simulink model "sixdof"  (Simulink 4.00)
settings: Solver=ode45  StartTime=0.0  StopTime=100  RelTol=1e-3
libraries: aerospace x3, simulink_extras x3, simulink3 x1
settings Model: Creator=mcar  LastModifiedBy=mcar  BlockReductionOpt=off

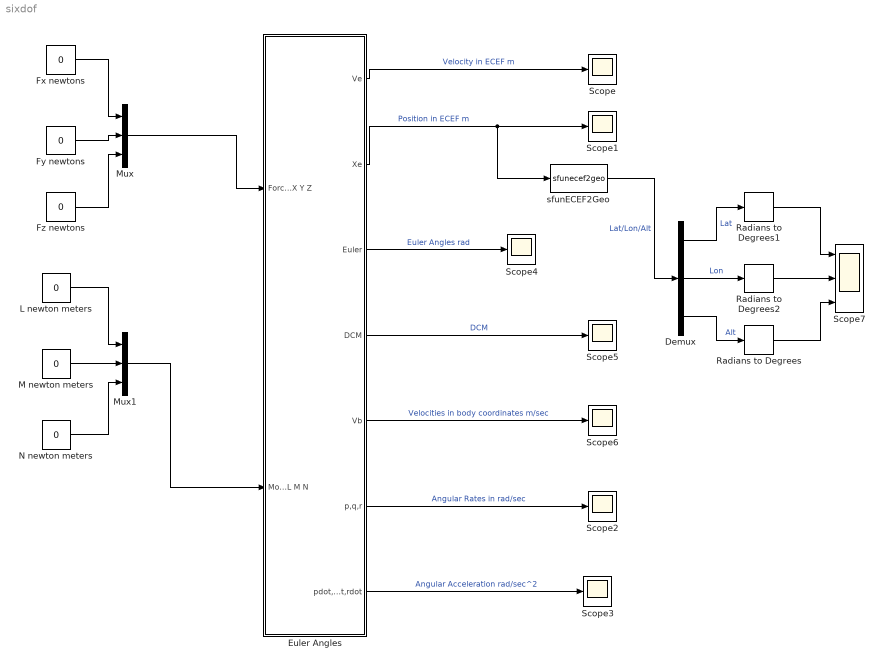
== system sixdof ==
  Demux : Demux  Outputs=3  BusSelectionMode=off
  Euler Angles : Subsystem  AncestorBlock=aerospace/6DoF/Euler Angles  mask{xme_0=[6.378137e6 0 0], Vm_0=[1 1 0], eul_0=[0 0 0], pm_0=[0 0 0], Mass=1.0, Inertia=[1.0 0 0;0 1.0 0;0 0 1.0]}
      mask prompts: xme_0 "Initial Inertial Position [Xe,Ye,Ze]"; Vm_0 "Initial Body Velocity [U,v,w]"; eul_0 "Initial Euler Orientation [roll, pitch, yaw]"; pm_0 "Initial Body Rates [p,q,r]"; Mass "Mass of body"; Inertia "Inertia Matrix"
      mask help: Euler Angles
      settings: RTWFcnNameOpts=Auto  RTWFileNameOpts=Auto
      mask Display: disp('Euler\nAngles')
  Fx newtons : Constant  Value=0
  Fy newtons : Constant  Value=0
  Fz newtons : Constant  Value=0
  L newton meters : Constant  Value=0
  M newton meters : Constant  Value=0
  Mux : Mux  Inputs=3
  Mux1 : Mux  Inputs=3
  N newton meters : Constant  Value=0
  Radians to Degrees : simulink_extras/Transformations/Radians to Degrees
  Radians to Degrees1 : simulink_extras/Transformations/Radians to Degrees
  Radians to Degrees2 : simulink_extras/Transformations/Radians to Degrees
  Scope{,1..6} (7 alike) : Scope
      Scope settings: TimeRange=auto  YMin=-5  YMax=5  SaveToWorkspace=off  SaveName=ScopeData  LimitDataPoints=on  MaxDataPoints=5000
      Scope1 settings: TickLabels=on  TimeRange=auto  YMin=-5  YMax=5  SaveToWorkspace=off  LimitDataPoints=on  MaxDataPoints=5000
      Scope2 settings: TimeRange=auto  YMin=-5  YMax=5  SaveToWorkspace=off  SaveName=ScopeData2  LimitDataPoints=on  MaxDataPoints=5000
      Scope3 settings: TimeRange=auto  YMin=-5  YMax=5  SaveToWorkspace=off  SaveName=ScopeData3  LimitDataPoints=on  MaxDataPoints=5000
      Scope4 settings: TickLabels=on  TimeRange=auto  YMin=-5  YMax=5  SaveToWorkspace=off  SaveName=ScopeData4  LimitDataPoints=on  MaxDataPoints=5000
      Scope5 settings: TickLabels=on  TimeRange=auto  YMin=-5  YMax=5  SaveToWorkspace=off  SaveName=ScopeData5  LimitDataPoints=on  MaxDataPoints=5000
      Scope6 settings: TickLabels=on  TimeRange=auto  YMin=-5  YMax=5  SaveToWorkspace=off  SaveName=ScopeData6  LimitDataPoints=on  MaxDataPoints=5000
  Scope7 : Scope  NumInputPorts=3
      settings: TickLabels=on  TimeRange=auto  YMin=-5~-5~-5  YMax=5~5~5  SaveToWorkspace=off  SaveName=ScopeData7  LimitDataPoints=on  MaxDataPoints=5000
  sfunECEF2Geo : S-Function  FunctionName=sfunecef2geo  PortCounts=[]  SFunctionModules=''
  wires:
  Mux/1 -> Euler Angles/1(Forces X Y Z)
  Fz newtons/1 -> Mux/3
  Fy newtons/1 -> Mux/2
  Fx newtons/1 -> Mux/1
  Mux1/1 -> Euler Angles/2(Moments L M N)
  N newton meters/1 -> Mux1/3
  M newton meters/1 -> Mux1/2
  L newton meters/1 -> Mux1/1
  Euler Angles/7(pdot,qdot,rdot) -> Scope3/1  "Angular Acceleration rad/sec^2"
  Euler Angles/6(p,q,r) -> Scope2/1  "Angular Rates in rad/sec"
  Euler Angles/2(Xe) -> Scope1/1, sfunECEF2Geo/1  "Position in ECEF m"
  Euler Angles/1(Ve) -> Scope/1  "Velocity in ECEF m"
  Euler Angles/3(Euler) -> Scope4/1  "Euler Angles rad"
  Euler Angles/5(Vb) -> Scope6/1  "Velocities in body coordinates m/sec"
  Euler Angles/4(DCM) -> Scope5/1  "DCM"
  sfunECEF2Geo/1 -> Demux/1  "Lat/Lon/Alt"
  Demux/1 -> Radians to Degrees1/1  "Lat"
  Demux/2 -> Radians to Degrees2/1  "Lon"
  Demux/3 -> Radians to Degrees/1  "Alt"
  Radians to Degrees1/1 -> Scope7/1
  Radians to Degrees2/1 -> Scope7/2
  Radians to Degrees/1 -> Scope7/3

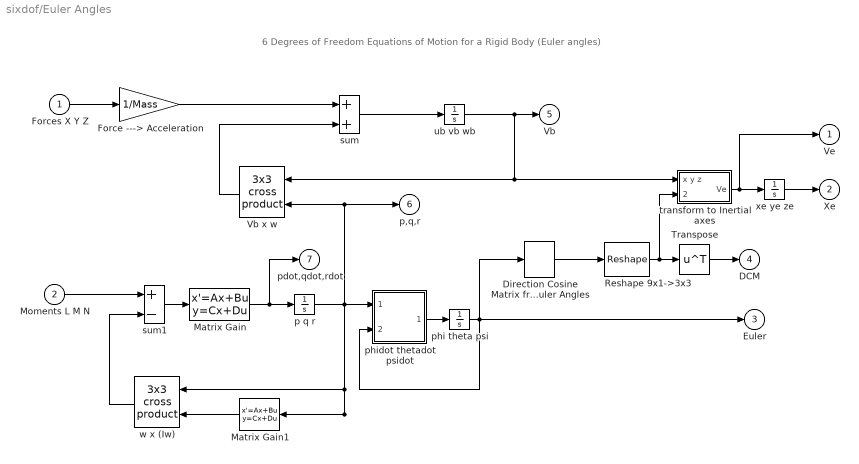
== system sixdof/Euler Angles ==
  note: 6 Degrees of Freedom Equations of Motion for a Rigid Body
      | (Euler angles)
  Forces X Y Z : Inport  Port=1
  Moments L M N : Inport  Port=2
  Direction Cosine Matrix from Euler Angles : aerospace/Axes Transformations/Direction Cosine Matrix from Euler Angles
  Force ---> Acceleration : Gain  Gain=1/Mass  Multiplication=Element-wise(K.*u)  SaturateOnIntegerOverflow=on
  Matrix Gain : StateSpace  A=[]  B=[]  C=[]  D=K  X0=0  Realization=auto  AbsoluteTolerance=auto  mask(Matrix Gain){@1=inv(Inertia)}
      mask prompts: @1 "Gain matrix:"
      mask help: Matrix Gain.
      mask init:
      | K = @1;
      mask Help: Multiplies input vector by entered matrix to produce output vector (y=Au).
      mask Display: disp('Inertia^(-1)')
  Matrix Gain1 : StateSpace  Orientation=left  A=[]  B=[]  C=[]  D=K  X0=0  Realization=auto  AbsoluteTolerance=auto  mask(Matrix Gain){@1=Inertia}
      mask prompts: @1 "Gain matrix:"
      mask help: Matrix Gain.
      mask init:
      | K = @1;
      mask Help: Multiplies input vector by entered matrix to produce output vector (y=Au).
      mask Display: disp('Inertia')
  Reshape 9x1->3x3 : simulink3/Signals & Systems/Reshape  OutputDimensionality=Customize  OutputDimensions=[3,3]
  Transpose : Math  Operator=transpose  OutputSignalType=auto
  Vb x w : aerospace/Axes Transformations/3x3 cross product  Orientation=left
  p q r : Integrator  ExternalReset=none  InitialConditionSource=internal  InitialCondition=pm_0  LimitOutput=off  UpperSaturationLimit=inf  LowerSaturationLimit=-inf  ShowSaturationPort=off  ShowStatePort=off  AbsoluteTolerance=auto
  phi theta psi : Integrator  ExternalReset=none  InitialConditionSource=internal  InitialCondition=eul_0  LimitOutput=off  UpperSaturationLimit=inf  LowerSaturationLimit=-inf  ShowSaturationPort=off  ShowStatePort=off  AbsoluteTolerance=auto
  phidot thetadot psidot : Subsystem
      settings: RTWFcnNameOpts=Auto  RTWFileNameOpts=Auto
  sum : Sum  Inputs=++  SaturateOnIntegerOverflow=on
  sum1 : Sum  Inputs=+-  SaturateOnIntegerOverflow=on
  "transform to Inertial axes " : Subsystem
      settings: RTWFcnNameOpts=Auto  RTWFileNameOpts=Auto
      mask Type: Vector Transformation
      mask Display: disp('L_EB')
  ub vb wb : Integrator  ExternalReset=none  InitialConditionSource=internal  InitialCondition=Vm_0  LimitOutput=off  UpperSaturationLimit=inf  LowerSaturationLimit=-inf  ShowSaturationPort=off  ShowStatePort=off  AbsoluteTolerance=auto
  w x (Iw) : aerospace/Axes Transformations/3x3 cross product  Orientation=left
  xe ye ze : Integrator  ExternalReset=none  InitialConditionSource=internal  InitialCondition=xme_0  LimitOutput=off  UpperSaturationLimit=inf  LowerSaturationLimit=-inf  ShowSaturationPort=off  ShowStatePort=off  AbsoluteTolerance=auto
  Ve : Outport  Port=1  InitialOutput=0
  Xe : Outport  Port=2  InitialOutput=0
  Euler : Outport  Port=3  InitialOutput=0
  DCM : Outport  Port=4  InitialOutput=0
  Vb : Outport  Port=5  InitialOutput=0
  p,q,r : Outport  Port=6  InitialOutput=0
  pdot,qdot,rdot : Outport  Port=7  InitialOutput=0
  wires:
  Transpose/1 -> DCM/1
  Reshape 9x1->3x3/1 -> Transpose/1, "transform to Inertial axes "/2(transform coefficients)
  Force ---> Acceleration/1 -> sum/1
  Vb x w/1 -> sum/2
  Forces X Y Z/1 -> Force ---> Acceleration/1
  Matrix Gain/1 -> pdot,qdot,rdot/1, p q r/1
  w x (Iw)/1 -> sum1/2
  Matrix Gain1/1 -> w x (Iw)/2
  Moments L M N/1 -> sum1/1
  sum1/1 -> Matrix Gain/1
  p q r/1 -> w x (Iw)/1, phidot thetadot psidot/1(p q r), Matrix Gain1/1, p,q,r/1, Vb x w/2
  "transform to Inertial axes "/1(Ve) -> Ve/1, xe ye ze/1
  xe ye ze/1 -> Xe/1
  sum/1 -> ub vb wb/1
  ub vb wb/1 -> "transform to Inertial axes "/1(x y z), Vb x w/1, Vb/1
  phi theta psi/1 -> phidot thetadot psidot/2(phi theta psi), Euler/1, Direction Cosine Matrix from Euler Angles/1
  phidot thetadot psidot/1(phidot thetadot psi) -> phi theta psi/1
  Direction Cosine Matrix from Euler Angles/1 -> Reshape 9x1->3x3/1

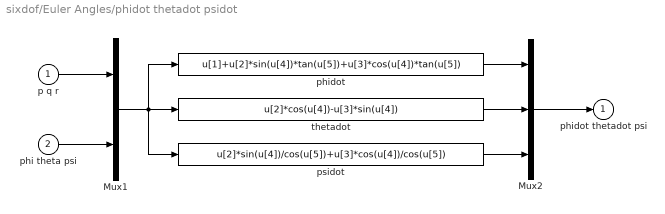
== system sixdof/Euler Angles/phidot thetadot psidot ==
  p q r : Inport  Port=1
  phi theta psi : Inport  Port=2
  Mux1 : Mux  Inputs=[3 3]
  Mux2 : Mux  Inputs=3
  phidot : Fcn  Expr=u[1]+u[2]*sin(u[4])*tan(u[5])+u[3]*cos(u[4])*tan(u[5])
  psidot : Fcn  Expr=u[2]*sin(u[4])/cos(u[5])+u[3]*cos(u[4])/cos(u[5])
  thetadot : Fcn  Expr=u[2]*cos(u[4])-u[3]*sin(u[4])
  phidot thetadot psi : Outport  Port=1  InitialOutput=0
  wires:
  Mux2/1 -> phidot thetadot psi/1
  phidot/1 -> Mux2/1
  thetadot/1 -> Mux2/2
  psidot/1 -> Mux2/3
  phi theta psi/1 -> Mux1/2
  p q r/1 -> Mux1/1
  Mux1/1 -> thetadot/1, phidot/1, psidot/1

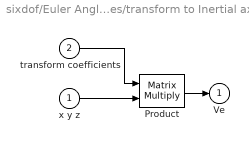
== system sixdof/Euler Angles/transform to Inertial axes  ==
  x y z : Inport  Port=1
  transform coefficients : Inport  Port=2
  Product : Product  Inputs=2  Multiplication=Matrix(*)  SaturateOnIntegerOverflow=on
  Ve : Outport  Port=1  InitialOutput=0
  wires:
  Product/1 -> Ve/1
  transform coefficients/1 -> Product/1
  x y z/1 -> Product/2
